simulink model "AvonGasTurbineFAult"  (R2016b)
settings: Solver=ode45  StartTime=0.0  StopTime=3000  FixedStep=1  RelTol=1e-3  EnableMultiTasking=on
InitFcn:
  | warning off
undefined symbols (not defined in the file or in its folder): flagFalut, thresholdbound, xflt
libraries: neural x74, fuzblock x6, simulink x5
(part 2 of 4)

== system AvonGasTurbineFAult/IGV/Layer 2 ==
  "a{1} " : Inport  PortDimensions=10
      mask Display: e = 0.06;c1 = [120 230 180]/255;c2 = ([120 230 180]+0)/(256+128);c3 = ([120 230 180]+128)/(256+128);patch([0 1 1 0],[0 0 1 1],c1);patch([0 1 1 1-e 1-e 0+e],[0 0 1 1-e 0+e 0+e],c2);patch([0 0 1 1-e 0+e 0+e],[0 1 1 1-e 1-e 0+e],c3);plot([0 1 1 0 0],[0 0 1 1 0]);
  Delays 1 : Subsystem
      mask Display: e = 0.06;c1 = [120 150 230]/255;c2 = ([120 150 230]+0)/383;c3 = ([120 150 230]+128)/383;patch([0 1 1 0],[0 0 1 1],c1);patch([0 1 1 1-e 1-e 0+e],[0 0 1 1-e 0+e 0+e],c2);patch([0 0 1 1-e 0+e 0+e],[0 1 1 1-e 1-e 0+e],c3);plot([0 1 1 0 0],[0 0 1 1 0]);disp('0');
  "LW{2,1}" : Subsystem
      mask Display: e = 0.06;c1 = [120 150 230]/255;c2 = ([120 150 230]+0)/383;c3 = ([120 150 230]+128)/383;patch([0 1 1 0],[0 0 1 1],c1);patch([0 1 1 1-e 1-e 0+e],[0 0 1 1-e 0+e 0+e],c2);patch([0 0 1 1-e 0+e 0+e],[0 1 1 1-e 1-e 0+e],c3);plot([0 1 1 0 0],[0 0 1 1 0]);disp('W');
  "b{2}" : Constant  Value=[-1.4853043976248173;-0.85618625825271266;-1.763034308041038;0.36633384062384799;1.9272762947772668]
      mask Display: e = 0.06;c1 = [120 150 230]/255;c2 = ([120 150 230]+0)/383;c3 = ([120 150 230]+128)/383;patch([0 1 1 0],[0 0 1 1],c1);patch([0 1 1 1-e 1-e 0+e],[0 0 1 1-e 0+e 0+e],c2);patch([0 0 1 1-e 0+e 0+e],[0 1 1 1-e 1-e 0+e],c3);plot([0 1 1 0 0],[0 0 1 1 0]);disp('b');
  netsum : Sum  Inputs=2  SaturateOnIntegerOverflow=on  InputSameDT=on  OutDataTypeStr=Inherit: Same as first input
      mask Display: e = 0.06;c1 = [120 150 230]/255;c2 = ([120 150 230]+0)/383;c3 = ([120 150 230]+128)/383;patch([0 1 1 0],[0 0 1 1],c1);patch([0 1 1 1-e 1-e 0+e],[0 0 1 1-e 0+e 0+e],c2);patch([0 0 1 1-e 0+e 0+e],[0 1 1 1-e 1-e 0+e],c3);plot([0 1 1 0 0],[0 0 1 1 0]);disp('+');
  softmax : neural/Transfer Functions/softmax
  "a{2}" : Outport  InitialOutput=[0;0;0;0;0]
      mask Display: e = 0.06;c1 = [120 230 180]/255;c2 = ([120 230 180]+0)/(256+128);c3 = ([120 230 180]+128)/(256+128);patch([0 1 1 0],[0 0 1 1],c1);patch([0 1 1 1-e 1-e 0+e],[0 0 1 1-e 0+e 0+e],c2);patch([0 0 1 1-e 0+e 0+e],[0 1 1 1-e 1-e 0+e],c3);plot([0 1 1 0 0],[0 0 1 1 0]);
  wires:
  "a{1} "/1 -> Delays 1/1("p{2}")
  Delays 1/1("pd{2,1}") -> "LW{2,1}"/1("ad{2,1}")
  "LW{2,1}"/1("lz{2,1}") -> netsum/1
  "b{2}"/1 -> netsum/2
  netsum/1 -> softmax/1
  softmax/1 -> "a{2}"/1

== system AvonGasTurbineFAult/IGV/Process Input 1 ==
  x : Inport  PortDimensions=6
      mask Display: e = 0.06;c1 = [120 230 180]/255;c2 = ([120 230 180]+0)/(256+128);c3 = ([120 230 180]+128)/(256+128);patch([0 1 1 0],[0 0 1 1],c1);patch([0 1 1 1-e 1-e 0+e],[0 0 1 1-e 0+e 0+e],c2);patch([0 0 1 1-e 0+e 0+e],[0 1 1 1-e 1-e 0+e],c3);plot([0 1 1 0 0],[0 0 1 1 0]);
  mapminmax : neural/Processing Functions/mapminmax  xmin=[-0.093008103798728925;0;-5.6896731350681762;0]  xmax=[0;20.262976664010012;-1.0691054727469123;22.645033295809071]  ymin=-1  ymax=1
  removeconstantrows : neural/Processing Functions/removeconstantrows  inputSize=6  keep=[1 3 4 5]
  p : Outport  PortDimensions=4
      mask Display: e = 0.06;c1 = [120 230 180]/255;c2 = ([120 230 180]+0)/(256+128);c3 = ([120 230 180]+128)/(256+128);patch([0 1 1 0],[0 0 1 1],c1);patch([0 1 1 1-e 1-e 0+e],[0 0 1 1-e 0+e 0+e],c2);patch([0 0 1 1-e 0+e 0+e],[0 1 1 1-e 1-e 0+e],c3);plot([0 1 1 0 0],[0 0 1 1 0]);
  wires:
  x/1 -> removeconstantrows/1
  removeconstantrows/1 -> mapminmax/1
  mapminmax/1 -> p/1

== system AvonGasTurbineFAult/IGV/Process Output 1 ==
  a : Inport  PortDimensions=5
      mask Display: e = 0.06;c1 = [120 230 180]/255;c2 = ([120 230 180]+0)/(256+128);c3 = ([120 230 180]+128)/(256+128);patch([0 1 1 0],[0 0 1 1],c1);patch([0 1 1 1-e 1-e 0+e],[0 0 1 1-e 0+e 0+e],c2);patch([0 0 1 1-e 0+e 0+e],[0 1 1 1-e 1-e 0+e],c3);plot([0 1 1 0 0],[0 0 1 1 0]);
  y : Outport  PortDimensions=5
      mask Display: e = 0.06;c1 = [120 230 180]/255;c2 = ([120 230 180]+0)/(256+128);c3 = ([120 230 180]+128)/(256+128);patch([0 1 1 0],[0 0 1 1],c1);patch([0 1 1 1-e 1-e 0+e],[0 0 1 1-e 0+e 0+e],c2);patch([0 0 1 1-e 0+e 0+e],[0 1 1 1-e 1-e 0+e],c3);plot([0 1 1 0 0],[0 0 1 1 0]);
  wires:
  a/1 -> y/1

== system AvonGasTurbineFAult/Subsystem/Combustor ==
  FG temp : Inport
  FG flow : Inport  Port=2
  FG press : Inport  Port=3
  air_flow : Inport  Port=4
  air temp : Inport  Port=5
  air_press : Inport  Port=6
  Scope1 : Scope
  Scope2 : Scope
  Scope3 : Scope
  combustion chamber 1 : Subsystem
  cooling_air_temp : Outport
  flow_chamber : Outport  Port=2
  temp_chamber : Outport  Port=3
  press_hot_gas : Outport  Port=4
  wires:
  FG flow/1 -> combustion chamber 1/1(Fg flow)
  FG press/1 -> combustion chamber 1/2(FG press)
  FG temp/1 -> combustion chamber 1/3(FG temp)
  combustion chamber 1/1(temp chamber 1) -> Scope1/1, temp_chamber/1
  air_press/1 -> combustion chamber 1/6(air_press)
  air temp/1 -> Scope2/1, cooling_air_temp/1, combustion chamber 1/5(air_temp)
  combustion chamber 1/2(flow) -> Scope3/1, flow_chamber/1
  air_flow/1 -> combustion chamber 1/4(air flow)
  combustion chamber 1/3(Gas_press) -> press_hot_gas/1

== system AvonGasTurbineFAult/Subsystem/FG MCV model ==
  FG CV pos (%) chmb1 : Inport
  main FG line prss : Inport  Port=2
  FG temp. : Inport  Port=3
  " Memory " : Memory  X0=1.9
  CV model chamber 2 : Subsystem
  Subsystem1 : Subsystem
  FG Temp (oC) : Outport
  FG Flow @bur (kg/s) : Outport  Port=2
  FG pr @bur (kPa) : Outport  Port=3
  FG skid inlet prss (kPa) : Outport  Port=4
  tag scope: FG_flow=global
  wires:
  Subsystem1/2(skid temp) -> CV model chamber 2/3(FG temp.)
  " Memory "/1 -> Subsystem1/3(FG flow)
  main FG line prss/1 -> Subsystem1/1(gas prss)
  Subsystem1/1(" FG skid inlet prss") -> CV model chamber 2/2(Skid inlet prss), FG skid inlet prss (kPa)/1
  FG temp./1 -> Subsystem1/2(FG temp.), FG Temp (oC)/1
  CV model chamber 2/1(FG pr @bur) -> FG pr @bur (kPa)/1
  FG CV pos (%) chmb1/1 -> CV model chamber 2/1(FG valve pos.)
  CV model chamber 2/2(FG flow) -> FG Flow @bur (kg/s)/1, [FG_flow], " Memory "/1

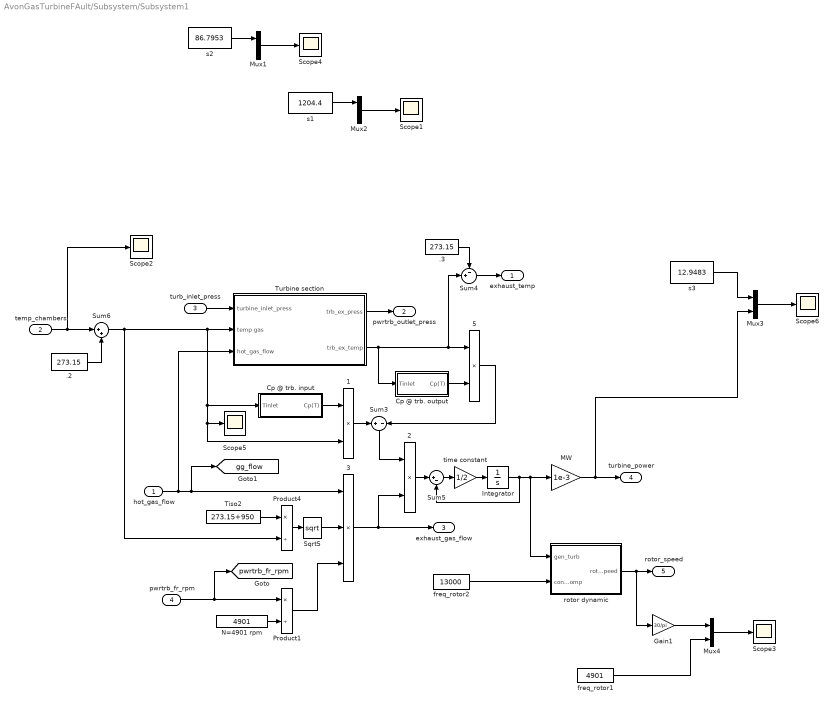
== system AvonGasTurbineFAult/Subsystem/Subsystem1 ==
  hot_gas_flow : Inport
  temp_chambers : Inport  Port=2
  turb_inlet_press : Inport  Port=3
  pwrtrb_fr_rpm : Inport  Port=4
  "    .2" : Constant  Value=273.15
  "    .3" : Constant  Value=273.15
  " 1" : Product  RndMeth=Zero
  " 2" : Product  RndMeth=Zero
  " 3" : Product  Inputs=3  RndMeth=Zero
  " 5" : Product  RndMeth=Zero
  Cp @ trb. input : Subsystem
  Cp @ trb. output : Subsystem
  Gain1 : Gain  Gain=30/pi
  Integrator : Integrator  InitialCondition=13000  LimitOutput=on  UpperSaturationLimit=20000  LowerSaturationLimit=1
  MW : Gain  Gain=1e-3
  Mux1 : Mux  Inputs=2
  Mux2 : Mux  Inputs=3
  Mux3 : Mux  Inputs=2
  Mux4 : Mux  Inputs=2
  N=4901 rpm : Constant  Value=4901
  Product1 : Product  Inputs=*/  RndMeth=Zero
  Product4 : Product  Inputs=*/  RndMeth=Zero
  Scope{1..6} (6 alike) : Scope
  Sqrt5 : Sqrt  SaturateOnIntegerOverflow=on
  Sum3 : Sum  Inputs=+-
  Sum4 : Sum  Inputs=-+|
  Sum5 : Sum  Inputs=|+-
  Sum6 : Sum  Inputs=|++
  Tiso2 : Constant  Value=273.15+950
  Turbine section : Subsystem
  freq_rotor1 : Constant  Value=4901
  freq_rotor2 : Constant  Value=13000
  rotor dynamic : Subsystem
  s1 : Constant  Value=1204.4
  s2 : Constant  Value=86.7953
  s3 : Constant  Value=12.9483
  time constant : Gain  Gain=1/2
  exhaust_temp : Outport
  pwrtrb_outlet_press : Outport  Port=2
  exhaust_gas_flow : Outport  Port=3
  turbine_power : Outport  Port=4
  rotor_speed : Outport  Port=5
  tag scope: gg_flow=global, pwrtrb_fr_rpm=global
  wires:
  Turbine section/2(trb_ex_temp) -> " 5"/1, Sum4/2, Cp @ trb. output/1(Tinlet)
  s3/1 -> Mux3/1
  Mux3/1 -> Scope6/1
  turb_inlet_press/1 -> Turbine section/1(turbine_inlet_press)
  "    .3"/1 -> Sum4/1
  Sum4/1 -> exhaust_temp/1
  temp_chambers/1 -> Scope2/1, Sum6/1
  "    .2"/1 -> Sum6/2
  s1/1 -> Mux2/1
  Mux2/1 -> Scope1/1
  s2/1 -> Mux1/1
  Mux1/1 -> Scope4/1
  " 2"/1 -> Sum5/1
  " 5"/1 -> Sum3/2
  Cp @ trb. output/1(Cp(T)) -> " 5"/2
  Cp @ trb. input/1(Cp(T)) -> " 1"/1
  time constant/1 -> Integrator/1
  Sum5/1 -> time constant/1
  " 1"/1 -> Sum3/1
  Sum3/1 -> " 2"/1
  Tiso2/1 -> Product4/1
  Sum6/1 -> Product4/2, Cp @ trb. input/1(Tinlet), " 1"/2, Scope5/1, Turbine section/2(temp gas)
  Product4/1 -> Sqrt5/1
  N=4901 rpm/1 -> Product1/2
  pwrtrb_fr_rpm/1 -> [pwrtrb_fr_rpm], Product1/1
  Product1/1 -> " 3"/3
  Sqrt5/1 -> " 3"/2
  hot_gas_flow/1 -> Turbine section/3(hot_gas_flow), [gg_flow], " 3"/1
  " 3"/1 -> exhaust_gas_flow/1, " 2"/2
  Turbine section/1(trb_ex_press) -> pwrtrb_outlet_press/1
  rotor dynamic/1(rotor_speed) -> Gain1/1, rotor_speed/1
  Integrator/1 -> Sum5/2, MW/1, rotor dynamic/1(gen_turb)
  MW/1 -> turbine_power/1, Mux3/2
  Mux4/1 -> Scope3/1
  freq_rotor1/1 -> Mux4/2
  Gain1/1 -> Mux4/1
  freq_rotor2/1 -> rotor dynamic/2(consm_comp)

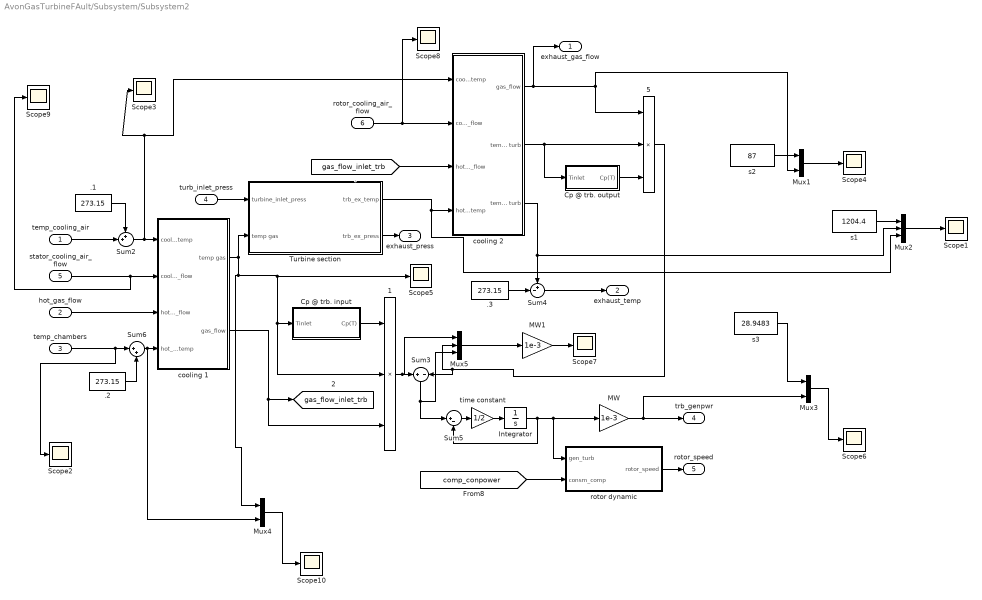
== system AvonGasTurbineFAult/Subsystem/Subsystem2 ==
  temp_cooling_air : Inport
  hot_gas_flow : Inport  Port=2
  temp_chambers : Inport  Port=3
  turb_inlet_press : Inport  Port=4
  stator_cooling_air_flow : Inport  Port=5
  rotor_cooling_air_flow : Inport  Port=6
  "    .1" : Constant  Value=273.15
  "    .2" : Constant  Value=273.15
  "    .3" : Constant  Value=273.15
  " 1" : Product  Inputs=3  RndMeth=Zero
  " 5" : Product  Inputs=3  RndMeth=Zero
  Cp @ trb. input : Subsystem
  Cp @ trb. output : Subsystem
  Integrator : Integrator  InitialCondition=13500  LimitOutput=on  UpperSaturationLimit=34000  LowerSaturationLimit=10
  MW : Gain  Gain=1e-3
  MW1 : Gain  Gain=1e-3
  Mux1 : Mux  Inputs=2
  Mux2 : Mux  Inputs=3
  Mux3 : Mux  Inputs=2
  Mux4 : Mux  Inputs=2
  Mux5 : Mux  Inputs=3
  Scope{1..10} (10 alike) : Scope
  Sum2 : Sum  Inputs=++|
  Sum3 : Sum  Inputs=+-
  Sum4 : Sum  Inputs=+-|
  Sum5 : Sum  Inputs=|+-
  Sum6 : Sum  Inputs=|++
  Turbine section : Subsystem
  cooling 1 : Subsystem
  cooling 2 : Subsystem
  "rotor dynamic " : Subsystem
  s1 : Constant  Value=1204.4
  s2 : Constant  Value=87
  s3 : Constant  Value=28.9483
  time constant : Gain  Gain=1/2
  exhaust_gas_flow : Outport
  exhaust_temp : Outport  Port=2
  exhaust_press : Outport  Port=3
  trb_genpwr : Outport  Port=4
  rotor_speed : Outport  Port=5
  tag scope: gas_flow_inlet_trb=global
  wires:
  Sum2/1 -> cooling 1/1(cooling_air_temp), cooling 2/1(cooling_air_temp), Scope3/1
  hot_gas_flow/1 -> cooling 1/3(hot_gas_flow)
  " 1"/1 -> Mux5/1, Sum3/1
  rotor_cooling_air_flow/1 -> Scope8/1, cooling 2/2(cooling_air_flow)
  Sum5/1 -> time constant/1
  time constant/1 -> Integrator/1
  [gas_flow_inlet_trb] -> cooling 2/3(hot_gas_flow)
  Cp @ trb. input/1(Cp(T)) -> " 1"/1
  Turbine section/1(trb_ex_temp) -> Mux2/3, cooling 2/4(hot_gas_temp)
  cooling 2/3(temp exh turb) -> Mux2/2, Sum4/1
  Cp @ trb. output/1(Cp(T)) -> " 5"/3
  " 5"/1 -> Sum3/2, Mux5/2
  cooling 1/2(gas_flow) -> " 1"/3, [gas_flow_inlet_trb]
  Sum3/1 -> Mux5/3, Sum5/1
  Mux1/1 -> Scope4/1
  s2/1 -> Mux1/1
  cooling 2/1(gas_flow) -> " 5"/1, Mux1/2, exhaust_gas_flow/1
  Mux2/1 -> Scope1/1
  s1/1 -> Mux2/1
  "    .1"/1 -> Sum2/1
  temp_cooling_air/1 -> Sum2/2
  "    .2"/1 -> Sum6/2
  temp_chambers/1 -> Scope2/1, Sum6/1
  Sum4/1 -> exhaust_temp/1
  "    .3"/1 -> Sum4/2
  turb_inlet_press/1 -> Turbine section/1(turbine_inlet_press)
  Mux3/1 -> Scope6/1
  s3/1 -> Mux3/1
  Integrator/1 -> "rotor dynamic "/1(gen_turb), MW/1, Sum5/2
  cooling 2/2(temp turb) -> Cp @ trb. output/1(Tinlet), " 5"/2
  Turbine section/2(trb_ex_press) -> exhaust_press/1
  MW/1 -> Mux3/2, trb_genpwr/1
  [comp_conpower] -> "rotor dynamic "/2(consm_comp)
  "rotor dynamic "/1(rotor_speed) -> rotor_speed/1
  stator_cooling_air_flow/1 -> cooling 1/2(cooling_air_flow), Scope9/1
  Mux4/1 -> Scope10/1
  cooling 1/1(temp gas) -> Turbine section/2(temp gas), Cp @ trb. input/1(Tinlet), " 1"/2, Scope5/1, Mux4/1
  Sum6/1 -> Mux4/2, cooling 1/4(hot_gas_temp)
  Mux5/1 -> MW1/1
  MW1/1 -> Scope7/1

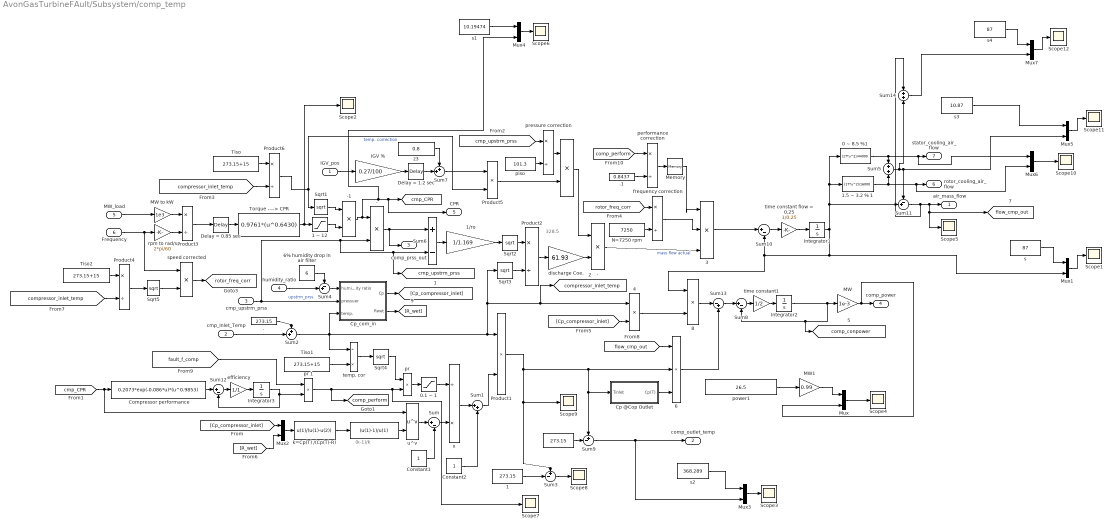
== system AvonGasTurbineFAult/Subsystem/comp_temp ==
  note: (k-1)/k
  note: 328.5
  IGV_pos : Inport
  cmp_Inlet_Temp : Inport  Port=2
  cmp_upstrm_prss : Inport  Port=3
  humidity_ratio : Inport  Port=4
  MW_load : Inport  Port=5
  Frequency : Inport  Port=6
  " " : Fcn  Expr=(u(1)-1)/u(1)
  "    " : Constant  Value=273.15
  "     " : Product  RndMeth=Zero
  "    1" : Constant  Value=273.15
  " 1.5 ~ 3.2 % 1" : Fcn  Expr=(17*u^2)/16000  SampleTime=1
  " 3" : Product  Inputs=3  RndMeth=Zero
  " 4" : Product  RndMeth=Zero
  " 6" : Product  Inputs=3  RndMeth=Zero
  " 8" : Product  RndMeth=Zero
  - : Product  RndMeth=Zero
  -1 : Product  RndMeth=Zero
  . : Constant  Value=273.15
  ". " : Product  RndMeth=Zero
  .1 : Constant  Value=0.8437
  0 ~ 8.5 %1 : Fcn  Expr=(17*u^2)/44000  SampleTime=1
  0.1 ~ 1 : Saturate  UpperLimit=1  LowerLimit=0.1
  1 ~ 12 : Saturate  UpperLimit=20  LowerLimit=1
  1/ro : Gain  Gain=1/1.169
  6% humidity drop in air filter : Constant  Value=6
  "Compressor performance " : Fcn  Expr=0.2073*exp(-0.086*u)*(u^0.9853)
  Constant1 : Constant
  Constant2 : Constant
  Cp @Cop Outlet : Subsystem
  Cp_com_in : Subsystem
  Delay = 0.85 sec : TransportDelay  DelayTime=0.85  InitialOutput=10.706
  Delay = 1.2 sec : TransportDelay  DelayTime=1.2  InitialOutput=0.27
  IGV % : Gain  Gain=0.27/100
  Integrator1 : Integrator  InitialCondition=87  LimitOutput=on  UpperSaturationLimit=140  LowerSaturationLimit=1
  Integrator2 : Integrator  InitialCondition=28000  LimitOutput=on  UpperSaturationLimit=32000  LowerSaturationLimit=10
  Integrator3 : Integrator  InitialCondition=0.6  LimitOutput=on  UpperSaturationLimit=1  LowerSaturationLimit=0
  MW : Gain  Gain=1e-3
  MW to kW : Gain  Gain=1e3
  MW1 : Gain  Gain=0.99
  Memory : Memory  X0=1.5
  Mux{,1..7} (8 alike) : Mux  Inputs=2
  N=7250 rpm : Constant  Value=7250
  Product1 : Product  RndMeth=Zero
  Product{2..4,6} (4 alike) : Product  Inputs=*/  RndMeth=Zero
  Product5 : Product  RndMeth=Zero
  Scope{1..12} (12 alike) : Scope
  Sqrt{1..5} (5 alike) : Sqrt  SaturateOnIntegerOverflow=on
  Sum{,8,10,12} (4 alike) : Sum  Inputs=|+-
  Sum1 : Sum  Inputs=|++
  Sum11 : Sum  Inputs=-+|
  Sum13 : Sum  Inputs=|-+
  Sum14 : Sum
  Sum2 : Sum  Inputs=++|
  Sum3 : Sum  Inputs=+-|
  Sum4 : Sum  Inputs=-+|
  Sum5 : Sum
  Sum6 : Sum  Inputs=+-
  Sum7 : Sum  Inputs=++|
  Sum9 : Sum  Inputs=+-|
  Tiso : Constant  Value=273.15+15
  Tiso1 : Constant  Value=273.15+15
  Tiso2 : Constant  Value=273.15+15
  Torque ----> CPR : Fcn  Expr=0.9761*(u^0.6430)
  "discharge Coe. " : Gain  Gain=61.93
  efficiency : Gain  Gain=1/1
  frequency correction : Product  Inputs=*/  RndMeth=Zero
  k=Cp(T) /(Cp(T)-R) : Fcn  Expr=u(1)/(u(1)-u(2))
  performance correction : Product  Inputs=*/  RndMeth=Zero
  piso : Constant  Value=101.3
  power1 : Constant  Value=26.5
  "pr " : Product  RndMeth=Zero
  pr 1 : Product  RndMeth=Zero
  pressure correction : Product  Inputs=*/  RndMeth=Zero
  rpm to rad/s : Gain  Gain=2*pi/60
  s : Constant  Value=87
  s1 : Constant  Value=10.19474
  s2 : Constant  Value=368.289
  s3 : Constant  Value=10.87
  s4 : Constant  Value=87
  speed corrected : Product  RndMeth=Zero
  temp. cor : Product  Inputs=/*  RndMeth=Zero
  time constant flow = 0.25 : Gain  Gain=1/0.25
  time constant1 : Gain  Gain=1/2
  u^v : Math  Operator=pow  SaturateOnIntegerOverflow=on
  x : Product  Inputs=/*  RndMeth=Zero
  z3 : Constant  Value=0.8
  air_mass_flow : Outport
  comp_outlet_temp : Outport  Port=2
  comp_prss_out : Outport  Port=3
  comp_power : Outport  Port=4
  CPR : Outport  Port=5
  rotor_cooling_air_flow : Outport  Port=6
  stator_cooling_air_flow : Outport  Port=7
  tag scope: cmp_CPR=global, cmp_upstrm_prss=global, comp_conpower=global, comp_perform=global, compressor_inlet_temp=global, flow_cmp_out=global, rotor_freq_corr=global
  wires:
  [cmp_CPR] -> "Compressor performance "/1, u^v/1
  " "/1 -> u^v/2
  u^v/1 -> Sum/1
  Sum/1 -> x/2
  Constant2/1 -> Sum1/2
  Sum1/1 -> Product1/2
  Sum2/1 -> Cp_com_in/3(temp.), Product1/1, Sqrt3/1, [compressor_inlet_temp], " 4"/1, temp. cor/1
  x/1 -> Sum1/1
  Constant1/1 -> Sum/2
  cmp_upstrm_prss/1 -> Cp_com_in/2(pressuer), -/2, Sum6/2, [cmp_upstrm_prss]  "upstrm_prss"
  cmp_Inlet_Temp/1 -> Sum2/2
  "Compressor performance "/1 -> Sum12/1
  0.1 ~ 1/1 -> x/1
  k=Cp(T) /(Cp(T)-R)/1 -> " "/1
  Cp_com_in/1(Cp) -> [Cp_compressor_inlet]
  Sum4/1 -> Cp_com_in/1(humidity ratio)
  humidity_ratio/1 -> Sum4/2
  6% humidity drop in air filter/1 -> Sum4/1
  -/1 -> comp_prss_out/1, Sum6/1
  Frequency/1 -> speed corrected/1, rpm to rad/s/1
  Sum6/1 -> 1/ro/1
  1/ro/1 -> Sqrt2/1
  Sqrt3/1 -> Product2/2
  Product2/1 -> "discharge Coe. "/1
  Sqrt2/1 -> Product2/1
  IGV_pos/1 -> IGV %/1
  piso/1 -> pressure correction/2
  [cmp_upstrm_prss] -> pressure correction/1
  Product5/1 -> "     "/2
  "discharge Coe. "/1 -> ". "/2
  "     "/1 -> ". "/1
  ". "/1 -> " 3"/3  "mass flow actual"
  Product6/1 -> Product5/2, Sqrt1/1  "temp. correction"
  Tiso/1 -> Product6/1
  [compressor_inlet_temp] -> Product6/2
  pressure correction/1 -> "     "/1
  1 ~ 12/1 -> -1/2
  N=7250 rpm/1 -> frequency correction/2
  [rotor_freq_corr] -> frequency correction/1
  frequency correction/1 -> " 3"/2
  " 3"/1 -> Sum10/1
  [Cp_compressor_inlet] -> " 4"/2
  Sum10/1 -> time constant flow = 0.25/1
  time constant flow = 0.25/1 -> Integrator1/1
  " 4"/1 -> " 8"/2
  " 8"/1 -> Sum13/1
  Sqrt1/1 -> -1/1
  Sum7/1 -> Product5/1
  z3/1 -> Sum7/1
  IGV %/1 -> Delay = 1.2 sec/1
  Delay = 1.2 sec/1 -> Sum7/2
  MW_load/1 -> MW to kW/1
  Cp_com_in/2(Rwet) -> [R_wet]
  Mux2/1 -> k=Cp(T) /(Cp(T)-R)/1
  [Cp_compressor_inlet] -> Mux2/1
  [R_wet] -> Mux2/2
  Sum8/1 -> time constant1/1
  time constant1/1 -> Integrator2/1
  Sum13/1 -> Sum8/1
  ./1 -> Sum2/1
  Tiso1/1 -> temp. cor/2
  temp. cor/1 -> Sqrt4/1
  "pr "/1 -> 0.1 ~ 1/1
  Sum12/1 -> efficiency/1
  efficiency/1 -> Integrator3/1
  Sqrt4/1 -> "pr "/1
  Torque ----> CPR/1 -> 1 ~ 12/1, Scope2/1
  MW to kW/1 -> Product3/1
  rpm to rad/s/1 -> Product3/2
  Integrator3/1 -> pr 1/2, Sum12/2
  Integrator2/1 -> MW/1, [comp_conpower], Sum8/2
  Product1/1 -> " 6"/2, Cp @Cop Outlet/1(Tinlet), Sum9/1, Scope9/1, Sum3/1
  Cp @Cop Outlet/1(Cp(T)) -> " 6"/3
  " 6"/1 -> Sum13/2
  "    "/1 -> Sum9/2
  Tiso2/1 -> Product4/1
  [compressor_inlet_temp] -> Product4/2
  speed corrected/1 -> [rotor_freq_corr]
  Product4/1 -> Sqrt5/1
  Sqrt5/1 -> speed corrected/2
  [flow_cmp_out] -> " 6"/1
  Mux/1 -> Scope4/1
  Sum11/1 -> Sum14/1, Scope5/1, [flow_cmp_out], air_mass_flow/1
  0 ~ 8.5 %1/1 -> Sum5/1, Mux6/1, stator_cooling_air_flow/1
  Integrator1/1 -> Mux1/2, " 8"/1, Sum10/2, Sum11/2, " 1.5 ~ 3.2 % 1"/1, 0 ~ 8.5 %1/1
  Mux1/1 -> Scope1/1
  s/1 -> Mux1/1
  Product3/1 -> Delay = 0.85 sec/1
  Delay = 0.85 sec/1 -> Torque ----> CPR/1
  power1/1 -> MW1/1
  Mux3/1 -> Scope3/1
  s2/1 -> Mux3/1
  MW/1 -> Mux/2, comp_power/1
  Mux4/1 -> Scope6/1
  s1/1 -> Mux4/1
  -1/1 -> -/1, Mux4/2, [cmp_CPR], CPR/1
  Sum9/1 -> Mux3/2, comp_outlet_temp/1
  "    1"/1 -> Sum3/2
  Sum3/1 -> Scope8/1
  MW1/1 -> Mux/1
  Sum5/1 -> Sum14/2, Sum11/1, Mux5/2
  Mux5/1 -> Scope11/1
  s3/1 -> Mux5/1
  Mux6/1 -> Scope10/1
  " 1.5 ~ 3.2 % 1"/1 -> Sum5/2, Mux6/2, rotor_cooling_air_flow/1
  Sum14/1 -> Mux7/2
  Mux7/1 -> Scope12/1
  s4/1 -> Mux7/1
  pr 1/1 -> [comp_perform], "pr "/2, Scope7/1
  [fault_f_comp] -> pr 1/1
  performance correction/1 -> Memory/1
  .1/1 -> performance correction/2
  [comp_perform] -> performance correction/1
  Memory/1 -> " 3"/1

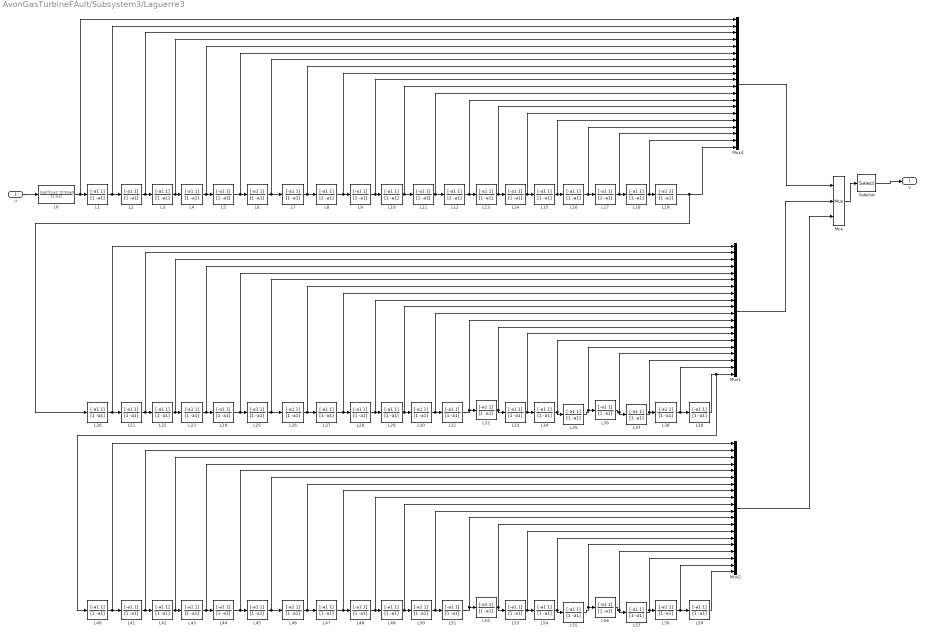
== system AvonGasTurbineFAult/Subsystem3/Laguerre3 ==
  u : Inport
  L0 : DiscreteTransferFcn  Numerator=[sqrt((1-a1^2)*smp)]  Denominator=[1 -a1]  SampleTime=smp  StateIdentifier=L0
  L{1..59} (59 alike) : DiscreteTransferFcn  Numerator=[-a1 1]  Denominator=[1 -a1]  SampleTime=smp  StateIdentifier=L1
  Mux : Mux  Inputs=3
  Mux1 : Mux  Inputs=20
  Mux2 : Mux  Inputs=20
  Mux4 : Mux  Inputs=20
  Selector : Selector  InputPortWidth=60  IndexOptions=Index vector (dialog)  Indices=1:fltrordr  OutputSizes=1
  v : Outport
  wires:
  Mux2/1 -> Mux/3
  L59/1 -> Mux2/20
  L58/1 -> L59/1, Mux2/19
  L57/1 -> L58/1, Mux2/18
  L56/1 -> L57/1, Mux2/17
  L55/1 -> L56/1, Mux2/16
  L54/1 -> L55/1, Mux2/15
  L53/1 -> L54/1, Mux2/14
  L52/1 -> L53/1, Mux2/13
  L51/1 -> L52/1, Mux2/12
  L50/1 -> L51/1, Mux2/11
  L49/1 -> L50/1, Mux2/10
  L48/1 -> L49/1, Mux2/9
  L47/1 -> L48/1, Mux2/8
  L46/1 -> L47/1, Mux2/7
  L45/1 -> L46/1, Mux2/6
  L44/1 -> L45/1, Mux2/5
  L43/1 -> L44/1, Mux2/4
  L42/1 -> L43/1, Mux2/3
  L41/1 -> L42/1, Mux2/2
  L40/1 -> L41/1, Mux2/1
  Selector/1 -> v/1
  Mux4/1 -> Mux/1
  Mux/1 -> Selector/1
  Mux1/1 -> Mux/2
  L39/1 -> Mux1/20, L40/1
  L38/1 -> Mux1/19, L39/1
  L37/1 -> Mux1/18, L38/1
  L36/1 -> Mux1/17, L37/1
  L35/1 -> Mux1/16, L36/1
  L34/1 -> Mux1/15, L35/1
  L33/1 -> Mux1/14, L34/1
  L32/1 -> Mux1/13, L33/1
  L31/1 -> Mux1/12, L32/1
  L30/1 -> Mux1/11, L31/1
  L29/1 -> Mux1/10, L30/1
  L28/1 -> Mux1/9, L29/1
  L27/1 -> Mux1/8, L28/1
  L26/1 -> Mux1/7, L27/1
  L25/1 -> Mux1/6, L26/1
  L24/1 -> Mux1/5, L25/1
  L23/1 -> Mux1/4, L24/1
  L22/1 -> Mux1/3, L23/1
  L21/1 -> Mux1/2, L22/1
  L20/1 -> Mux1/1, L21/1
  L19/1 -> L20/1, Mux4/20
  L18/1 -> Mux4/19, L19/1
  L17/1 -> Mux4/18, L18/1
  L16/1 -> Mux4/17, L17/1
  L15/1 -> Mux4/16, L16/1
  L14/1 -> Mux4/15, L15/1
  L13/1 -> Mux4/14, L14/1
  L12/1 -> Mux4/13, L13/1
  L11/1 -> Mux4/12, L12/1
  L10/1 -> Mux4/11, L11/1
  L9/1 -> Mux4/10, L10/1
  L8/1 -> Mux4/9, L9/1
  u/1 -> L0/1
  L7/1 -> Mux4/8, L8/1
  L6/1 -> L7/1, Mux4/7
  L5/1 -> L6/1, Mux4/6
  L0/1 -> Mux4/1, L1/1
  L4/1 -> L5/1, Mux4/5
  L3/1 -> L4/1, Mux4/4
  L2/1 -> L3/1, Mux4/3
  L1/1 -> L2/1, Mux4/2

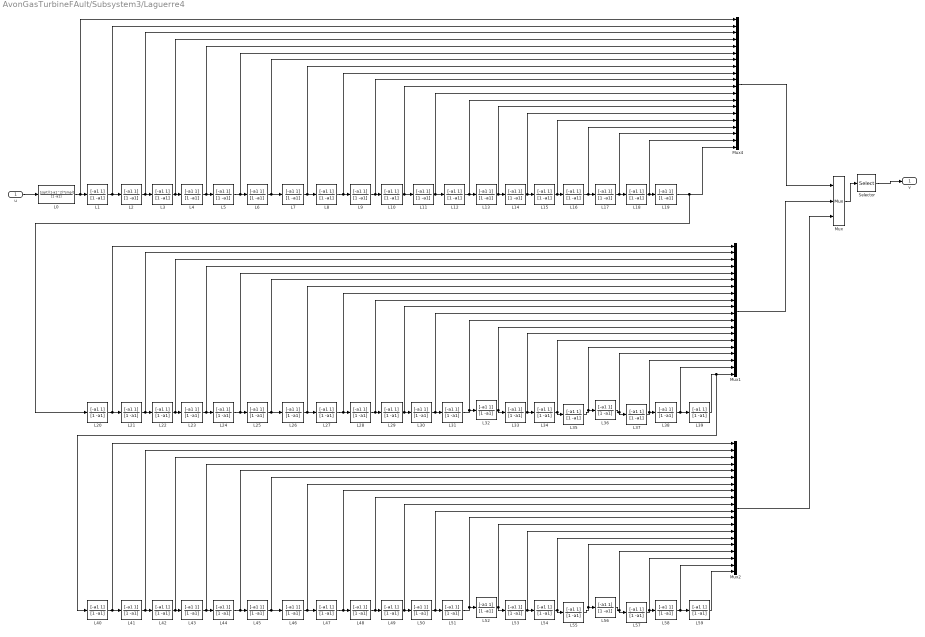
== system AvonGasTurbineFAult/Subsystem3/Laguerre4 ==
  u : Inport
  L0 : DiscreteTransferFcn  Numerator=[sqrt((1-a1^2)*smp)]  Denominator=[1 -a1]  SampleTime=smp  StateIdentifier=L0
  L{1..59} (59 alike) : DiscreteTransferFcn  Numerator=[-a1 1]  Denominator=[1 -a1]  SampleTime=smp  StateIdentifier=L1
  Mux : Mux  Inputs=3
  Mux1 : Mux  Inputs=20
  Mux2 : Mux  Inputs=20
  Mux4 : Mux  Inputs=20
  Selector : Selector  InputPortWidth=60  IndexOptions=Index vector (dialog)  Indices=1:fltrordr  OutputSizes=1
  v : Outport
  wires:
  L1/1 -> Mux4/2, L2/1
  L2/1 -> Mux4/3, L3/1
  L3/1 -> Mux4/4, L4/1
  L4/1 -> Mux4/5, L5/1
  L0/1 -> L1/1, Mux4/1
  L5/1 -> Mux4/6, L6/1
  L6/1 -> Mux4/7, L7/1
  L7/1 -> L8/1, Mux4/8
  u/1 -> L0/1
  L8/1 -> L9/1, Mux4/9
  L9/1 -> L10/1, Mux4/10
  L10/1 -> L11/1, Mux4/11
  L11/1 -> L12/1, Mux4/12
  L12/1 -> L13/1, Mux4/13
  L13/1 -> L14/1, Mux4/14
  L14/1 -> L15/1, Mux4/15
  L15/1 -> L16/1, Mux4/16
  L16/1 -> L17/1, Mux4/17
  L17/1 -> L18/1, Mux4/18
  L18/1 -> L19/1, Mux4/19
  L19/1 -> Mux4/20, L20/1
  L20/1 -> L21/1, Mux1/1
  L21/1 -> L22/1, Mux1/2
  L22/1 -> L23/1, Mux1/3
  L23/1 -> L24/1, Mux1/4
  L24/1 -> L25/1, Mux1/5
  L25/1 -> L26/1, Mux1/6
  L26/1 -> L27/1, Mux1/7
  L27/1 -> L28/1, Mux1/8
  L28/1 -> L29/1, Mux1/9
  L29/1 -> L30/1, Mux1/10
  L30/1 -> L31/1, Mux1/11
  L31/1 -> L32/1, Mux1/12
  L32/1 -> L33/1, Mux1/13
  L33/1 -> L34/1, Mux1/14
  L34/1 -> L35/1, Mux1/15
  L35/1 -> L36/1, Mux1/16
  L36/1 -> L37/1, Mux1/17
  L37/1 -> L38/1, Mux1/18
  L38/1 -> L39/1, Mux1/19
  L39/1 -> L40/1, Mux1/20
  Mux1/1 -> Mux/2
  Mux/1 -> Selector/1
  Mux4/1 -> Mux/1
  Selector/1 -> v/1
  L40/1 -> Mux2/1, L41/1
  L41/1 -> Mux2/2, L42/1
  L42/1 -> Mux2/3, L43/1
  L43/1 -> Mux2/4, L44/1
  L44/1 -> Mux2/5, L45/1
  L45/1 -> Mux2/6, L46/1
  L46/1 -> Mux2/7, L47/1
  L47/1 -> Mux2/8, L48/1
  L48/1 -> Mux2/9, L49/1
  L49/1 -> Mux2/10, L50/1
  L50/1 -> Mux2/11, L51/1
  L51/1 -> Mux2/12, L52/1
  L52/1 -> Mux2/13, L53/1
  L53/1 -> Mux2/14, L54/1
  L54/1 -> Mux2/15, L55/1
  L55/1 -> Mux2/16, L56/1
  L56/1 -> Mux2/17, L57/1
  L57/1 -> Mux2/18, L58/1
  L58/1 -> Mux2/19, L59/1
  L59/1 -> Mux2/20
  Mux2/1 -> Mux/3

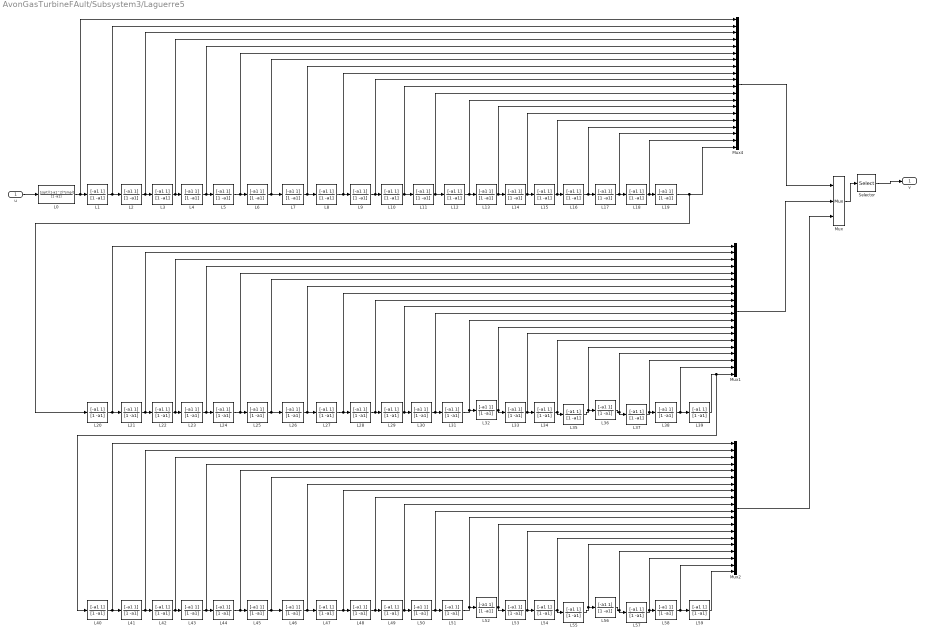
== system AvonGasTurbineFAult/Subsystem3/Laguerre5 ==
  u : Inport
  L0 : DiscreteTransferFcn  Numerator=[sqrt((1-a1^2)*smp)]  Denominator=[1 -a1]  SampleTime=smp  StateIdentifier=L0
  L{1..59} (59 alike) : DiscreteTransferFcn  Numerator=[-a1 1]  Denominator=[1 -a1]  SampleTime=smp  StateIdentifier=L1
  Mux : Mux  Inputs=3
  Mux1 : Mux  Inputs=20
  Mux2 : Mux  Inputs=20
  Mux4 : Mux  Inputs=20
  Selector : Selector  InputPortWidth=60  IndexOptions=Index vector (dialog)  Indices=1:fltrordr  OutputSizes=1
  v : Outport
  wires:
  Mux2/1 -> Mux/3
  L59/1 -> Mux2/20
  L58/1 -> L59/1, Mux2/19
  L57/1 -> L58/1, Mux2/18
  L56/1 -> L57/1, Mux2/17
  L55/1 -> L56/1, Mux2/16
  L54/1 -> L55/1, Mux2/15
  L53/1 -> L54/1, Mux2/14
  L52/1 -> L53/1, Mux2/13
  L51/1 -> L52/1, Mux2/12
  L50/1 -> L51/1, Mux2/11
  L49/1 -> L50/1, Mux2/10
  L48/1 -> L49/1, Mux2/9
  L47/1 -> L48/1, Mux2/8
  L46/1 -> L47/1, Mux2/7
  L45/1 -> L46/1, Mux2/6
  L44/1 -> L45/1, Mux2/5
  L43/1 -> L44/1, Mux2/4
  L42/1 -> L43/1, Mux2/3
  L41/1 -> L42/1, Mux2/2
  L40/1 -> L41/1, Mux2/1
  Selector/1 -> v/1
  Mux4/1 -> Mux/1
  Mux/1 -> Selector/1
  Mux1/1 -> Mux/2
  L39/1 -> Mux1/20, L40/1
  L38/1 -> Mux1/19, L39/1
  L37/1 -> Mux1/18, L38/1
  L36/1 -> Mux1/17, L37/1
  L35/1 -> Mux1/16, L36/1
  L34/1 -> Mux1/15, L35/1
  L33/1 -> Mux1/14, L34/1
  L32/1 -> Mux1/13, L33/1
  L31/1 -> Mux1/12, L32/1
  L30/1 -> Mux1/11, L31/1
  L29/1 -> Mux1/10, L30/1
  L28/1 -> Mux1/9, L29/1
  L27/1 -> Mux1/8, L28/1
  L26/1 -> Mux1/7, L27/1
  L25/1 -> Mux1/6, L26/1
  L24/1 -> Mux1/5, L25/1
  L23/1 -> Mux1/4, L24/1
  L22/1 -> Mux1/3, L23/1
  L21/1 -> Mux1/2, L22/1
  L20/1 -> Mux1/1, L21/1
  L19/1 -> L20/1, Mux4/20
  L18/1 -> Mux4/19, L19/1
  L17/1 -> Mux4/18, L18/1
  L16/1 -> Mux4/17, L17/1
  L15/1 -> Mux4/16, L16/1
  L14/1 -> Mux4/15, L15/1
  L13/1 -> Mux4/14, L14/1
  L12/1 -> Mux4/13, L13/1
  L11/1 -> Mux4/12, L12/1
  L10/1 -> Mux4/11, L11/1
  L9/1 -> Mux4/10, L10/1
  L8/1 -> Mux4/9, L9/1
  u/1 -> L0/1
  L7/1 -> Mux4/8, L8/1
  L6/1 -> L7/1, Mux4/7
  L5/1 -> L6/1, Mux4/6
  L0/1 -> Mux4/1, L1/1
  L4/1 -> L5/1, Mux4/5
  L3/1 -> L4/1, Mux4/4
  L2/1 -> L3/1, Mux4/3
  L1/1 -> L2/1, Mux4/2

== system AvonGasTurbineFAult/comp performance/Layer 1 ==
  "p{1}" : Inport  PortDimensions=6
      mask Display: e = 0.06;c1 = [120 230 180]/255;c2 = ([120 230 180]+0)/(256+128);c3 = ([120 230 180]+128)/(256+128);patch([0 1 1 0],[0 0 1 1],c1);patch([0 1 1 1-e 1-e 0+e],[0 0 1 1-e 0+e 0+e],c2);patch([0 0 1 1-e 0+e 0+e],[0 1 1 1-e 1-e 0+e],c3);plot([0 1 1 0 0],[0 0 1 1 0]);
  Delays 1 : Subsystem
      mask Display: e = 0.06;c1 = [120 150 230]/255;c2 = ([120 150 230]+0)/383;c3 = ([120 150 230]+128)/383;patch([0 1 1 0],[0 0 1 1],c1);patch([0 1 1 1-e 1-e 0+e],[0 0 1 1-e 0+e 0+e],c2);patch([0 0 1 1-e 0+e 0+e],[0 1 1 1-e 1-e 0+e],c3);plot([0 1 1 0 0],[0 0 1 1 0]);disp('0');
  "IW{1,1}" : Subsystem
      mask Display: e = 0.06;c1 = [120 150 230]/255;c2 = ([120 150 230]+0)/383;c3 = ([120 150 230]+128)/383;patch([0 1 1 0],[0 0 1 1],c1);patch([0 1 1 1-e 1-e 0+e],[0 0 1 1-e 0+e 0+e],c2);patch([0 0 1 1-e 0+e 0+e],[0 1 1 1-e 1-e 0+e],c3);plot([0 1 1 0 0],[0 0 1 1 0]);disp('W');
  "b{1}" : Constant  Value=[-3.0166662633594057;1.0701809085177809;-1.6446607077141964;-0.55262743191566366;0.81692339434643979;-0.80237414732459966;0.76663591739284342;0.41098680957882483;-2.2933622794585817;-2.2588966761883844]
      mask Display: e = 0.06;c1 = [120 150 230]/255;c2 = ([120 150 230]+0)/383;c3 = ([120 150 230]+128)/383;patch([0 1 1 0],[0 0 1 1],c1);patch([0 1 1 1-e 1-e 0+e],[0 0 1 1-e 0+e 0+e],c2);patch([0 0 1 1-e 0+e 0+e],[0 1 1 1-e 1-e 0+e],c3);plot([0 1 1 0 0],[0 0 1 1 0]);disp('b');
  netsum : Sum  Inputs=2  SaturateOnIntegerOverflow=on  InputSameDT=on  OutDataTypeStr=Inherit: Same as first input
      mask Display: e = 0.06;c1 = [120 150 230]/255;c2 = ([120 150 230]+0)/383;c3 = ([120 150 230]+128)/383;patch([0 1 1 0],[0 0 1 1],c1);patch([0 1 1 1-e 1-e 0+e],[0 0 1 1-e 0+e 0+e],c2);patch([0 0 1 1-e 0+e 0+e],[0 1 1 1-e 1-e 0+e],c3);plot([0 1 1 0 0],[0 0 1 1 0]);disp('+');
  tansig : neural/Transfer Functions/tansig
  "a{1}" : Outport  InitialOutput=[0;0;0;0;0;0;0;0;0;0]
      mask Display: e = 0.06;c1 = [120 230 180]/255;c2 = ([120 230 180]+0)/(256+128);c3 = ([120 230 180]+128)/(256+128);patch([0 1 1 0],[0 0 1 1],c1);patch([0 1 1 1-e 1-e 0+e],[0 0 1 1-e 0+e 0+e],c2);patch([0 0 1 1-e 0+e 0+e],[0 1 1 1-e 1-e 0+e],c3);plot([0 1 1 0 0],[0 0 1 1 0]);
  wires:
  "p{1}"/1 -> Delays 1/1("p{1}")
  Delays 1/1("pd{1,1}") -> "IW{1,1}"/1("pd{1,1}")
  "IW{1,1}"/1("iz{1,1}") -> netsum/1
  "b{1}"/1 -> netsum/2
  netsum/1 -> tansig/1
  tansig/1 -> "a{1}"/1

== system AvonGasTurbineFAult/comp performance/Layer 2 ==
  "a{1} " : Inport  PortDimensions=10
      mask Display: e = 0.06;c1 = [120 230 180]/255;c2 = ([120 230 180]+0)/(256+128);c3 = ([120 230 180]+128)/(256+128);patch([0 1 1 0],[0 0 1 1],c1);patch([0 1 1 1-e 1-e 0+e],[0 0 1 1-e 0+e 0+e],c2);patch([0 0 1 1-e 0+e 0+e],[0 1 1 1-e 1-e 0+e],c3);plot([0 1 1 0 0],[0 0 1 1 0]);
  Delays 1 : Subsystem
      mask Display: e = 0.06;c1 = [120 150 230]/255;c2 = ([120 150 230]+0)/383;c3 = ([120 150 230]+128)/383;patch([0 1 1 0],[0 0 1 1],c1);patch([0 1 1 1-e 1-e 0+e],[0 0 1 1-e 0+e 0+e],c2);patch([0 0 1 1-e 0+e 0+e],[0 1 1 1-e 1-e 0+e],c3);plot([0 1 1 0 0],[0 0 1 1 0]);disp('0');
  "LW{2,1}" : Subsystem
      mask Display: e = 0.06;c1 = [120 150 230]/255;c2 = ([120 150 230]+0)/383;c3 = ([120 150 230]+128)/383;patch([0 1 1 0],[0 0 1 1],c1);patch([0 1 1 1-e 1-e 0+e],[0 0 1 1-e 0+e 0+e],c2);patch([0 0 1 1-e 0+e 0+e],[0 1 1 1-e 1-e 0+e],c3);plot([0 1 1 0 0],[0 0 1 1 0]);disp('W');
  "b{2}" : Constant  Value=[-1.7513533865709121;-0.36843921322469791;0.099194300057818097;0.34826117446019883;3.3782784836596536]
      mask Display: e = 0.06;c1 = [120 150 230]/255;c2 = ([120 150 230]+0)/383;c3 = ([120 150 230]+128)/383;patch([0 1 1 0],[0 0 1 1],c1);patch([0 1 1 1-e 1-e 0+e],[0 0 1 1-e 0+e 0+e],c2);patch([0 0 1 1-e 0+e 0+e],[0 1 1 1-e 1-e 0+e],c3);plot([0 1 1 0 0],[0 0 1 1 0]);disp('b');
  netsum : Sum  Inputs=2  SaturateOnIntegerOverflow=on  InputSameDT=on  OutDataTypeStr=Inherit: Same as first input
      mask Display: e = 0.06;c1 = [120 150 230]/255;c2 = ([120 150 230]+0)/383;c3 = ([120 150 230]+128)/383;patch([0 1 1 0],[0 0 1 1],c1);patch([0 1 1 1-e 1-e 0+e],[0 0 1 1-e 0+e 0+e],c2);patch([0 0 1 1-e 0+e 0+e],[0 1 1 1-e 1-e 0+e],c3);plot([0 1 1 0 0],[0 0 1 1 0]);disp('+');
  softmax : neural/Transfer Functions/softmax
  "a{2}" : Outport  InitialOutput=[0;0;0;0;0]
      mask Display: e = 0.06;c1 = [120 230 180]/255;c2 = ([120 230 180]+0)/(256+128);c3 = ([120 230 180]+128)/(256+128);patch([0 1 1 0],[0 0 1 1],c1);patch([0 1 1 1-e 1-e 0+e],[0 0 1 1-e 0+e 0+e],c2);patch([0 0 1 1-e 0+e 0+e],[0 1 1 1-e 1-e 0+e],c3);plot([0 1 1 0 0],[0 0 1 1 0]);
  wires:
  "a{1} "/1 -> Delays 1/1("p{2}")
  Delays 1/1("pd{2,1}") -> "LW{2,1}"/1("ad{2,1}")
  "LW{2,1}"/1("lz{2,1}") -> netsum/1
  "b{2}"/1 -> netsum/2
  netsum/1 -> softmax/1
  softmax/1 -> "a{2}"/1

== system AvonGasTurbineFAult/comp performance/Process Input 1 ==
  x : Inport  PortDimensions=6
      mask Display: e = 0.06;c1 = [120 230 180]/255;c2 = ([120 230 180]+0)/(256+128);c3 = ([120 230 180]+128)/(256+128);patch([0 1 1 0],[0 0 1 1],c1);patch([0 1 1 1-e 1-e 0+e],[0 0 1 1-e 0+e 0+e],c2);patch([0 0 1 1-e 0+e 0+e],[0 1 1 1-e 1-e 0+e],c3);plot([0 1 1 0 0],[0 0 1 1 0]);
  mapminmax : neural/Processing Functions/mapminmax  xmin=[-0.0099251436812934912;0;0;-2.7206457077544428;0;0]  xmax=[0.37230275618354725;62.920409543555763;26.300756094012741;13.627941217339298;30.663666242441877;1.0233056862835035]  ymin=-1  ymax=1
  p : Outport  PortDimensions=6
      mask Display: e = 0.06;c1 = [120 230 180]/255;c2 = ([120 230 180]+0)/(256+128);c3 = ([120 230 180]+128)/(256+128);patch([0 1 1 0],[0 0 1 1],c1);patch([0 1 1 1-e 1-e 0+e],[0 0 1 1-e 0+e 0+e],c2);patch([0 0 1 1-e 0+e 0+e],[0 1 1 1-e 1-e 0+e],c3);plot([0 1 1 0 0],[0 0 1 1 0]);
  wires:
  x/1 -> mapminmax/1
  mapminmax/1 -> p/1

== system AvonGasTurbineFAult/comp performance/Process Output 1 ==
  a : Inport  PortDimensions=5
      mask Display: e = 0.06;c1 = [120 230 180]/255;c2 = ([120 230 180]+0)/(256+128);c3 = ([120 230 180]+128)/(256+128);patch([0 1 1 0],[0 0 1 1],c1);patch([0 1 1 1-e 1-e 0+e],[0 0 1 1-e 0+e 0+e],c2);patch([0 0 1 1-e 0+e 0+e],[0 1 1 1-e 1-e 0+e],c3);plot([0 1 1 0 0],[0 0 1 1 0]);
  y : Outport  PortDimensions=5
      mask Display: e = 0.06;c1 = [120 230 180]/255;c2 = ([120 230 180]+0)/(256+128);c3 = ([120 230 180]+128)/(256+128);patch([0 1 1 0],[0 0 1 1],c1);patch([0 1 1 1-e 1-e 0+e],[0 0 1 1-e 0+e 0+e],c2);patch([0 0 1 1-e 0+e 0+e],[0 1 1 1-e 1-e 0+e],c3);plot([0 1 1 0 0],[0 0 1 1 0]);
  wires:
  a/1 -> y/1

== system AvonGasTurbineFAult/exhst temp turbine gg/Layer 1 ==
  "p{1}" : Inport  PortDimensions=4
      mask Display: e = 0.06;c1 = [120 230 180]/255;c2 = ([120 230 180]+0)/(256+128);c3 = ([120 230 180]+128)/(256+128);patch([0 1 1 0],[0 0 1 1],c1);patch([0 1 1 1-e 1-e 0+e],[0 0 1 1-e 0+e 0+e],c2);patch([0 0 1 1-e 0+e 0+e],[0 1 1 1-e 1-e 0+e],c3);plot([0 1 1 0 0],[0 0 1 1 0]);
  Delays 1 : Subsystem
      mask Display: e = 0.06;c1 = [120 150 230]/255;c2 = ([120 150 230]+0)/383;c3 = ([120 150 230]+128)/383;patch([0 1 1 0],[0 0 1 1],c1);patch([0 1 1 1-e 1-e 0+e],[0 0 1 1-e 0+e 0+e],c2);patch([0 0 1 1-e 0+e 0+e],[0 1 1 1-e 1-e 0+e],c3);plot([0 1 1 0 0],[0 0 1 1 0]);disp('0');
  "IW{1,1}" : Subsystem
      mask Display: e = 0.06;c1 = [120 150 230]/255;c2 = ([120 150 230]+0)/383;c3 = ([120 150 230]+128)/383;patch([0 1 1 0],[0 0 1 1],c1);patch([0 1 1 1-e 1-e 0+e],[0 0 1 1-e 0+e 0+e],c2);patch([0 0 1 1-e 0+e 0+e],[0 1 1 1-e 1-e 0+e],c3);plot([0 1 1 0 0],[0 0 1 1 0]);disp('W');
  "b{1}" : Constant  Value=[-0.36714433505719574;4.171957052168457;-1.7610679720239906;2.1955821867065644;-1.7361627653117517;0.89571232552353919;-3.7724969892838036;-1.4077208997705311;3.1301228479901151;-1.435337158107306]
      mask Display: e = 0.06;c1 = [120 150 230]/255;c2 = ([120 150 230]+0)/383;c3 = ([120 150 230]+128)/383;patch([0 1 1 0],[0 0 1 1],c1);patch([0 1 1 1-e 1-e 0+e],[0 0 1 1-e 0+e 0+e],c2);patch([0 0 1 1-e 0+e 0+e],[0 1 1 1-e 1-e 0+e],c3);plot([0 1 1 0 0],[0 0 1 1 0]);disp('b');
  netsum : Sum  Inputs=2  SaturateOnIntegerOverflow=on  InputSameDT=on  OutDataTypeStr=Inherit: Same as first input
      mask Display: e = 0.06;c1 = [120 150 230]/255;c2 = ([120 150 230]+0)/383;c3 = ([120 150 230]+128)/383;patch([0 1 1 0],[0 0 1 1],c1);patch([0 1 1 1-e 1-e 0+e],[0 0 1 1-e 0+e 0+e],c2);patch([0 0 1 1-e 0+e 0+e],[0 1 1 1-e 1-e 0+e],c3);plot([0 1 1 0 0],[0 0 1 1 0]);disp('+');
  tansig : neural/Transfer Functions/tansig
  "a{1}" : Outport  InitialOutput=[0;0;0;0;0;0;0;0;0;0]
      mask Display: e = 0.06;c1 = [120 230 180]/255;c2 = ([120 230 180]+0)/(256+128);c3 = ([120 230 180]+128)/(256+128);patch([0 1 1 0],[0 0 1 1],c1);patch([0 1 1 1-e 1-e 0+e],[0 0 1 1-e 0+e 0+e],c2);patch([0 0 1 1-e 0+e 0+e],[0 1 1 1-e 1-e 0+e],c3);plot([0 1 1 0 0],[0 0 1 1 0]);
  wires:
  "p{1}"/1 -> Delays 1/1("p{1}")
  Delays 1/1("pd{1,1}") -> "IW{1,1}"/1("pd{1,1}")
  "IW{1,1}"/1("iz{1,1}") -> netsum/1
  "b{1}"/1 -> netsum/2
  netsum/1 -> tansig/1
  tansig/1 -> "a{1}"/1

== system AvonGasTurbineFAult/exhst temp turbine gg/Layer 2 ==
  "a{1} " : Inport  PortDimensions=10
      mask Display: e = 0.06;c1 = [120 230 180]/255;c2 = ([120 230 180]+0)/(256+128);c3 = ([120 230 180]+128)/(256+128);patch([0 1 1 0],[0 0 1 1],c1);patch([0 1 1 1-e 1-e 0+e],[0 0 1 1-e 0+e 0+e],c2);patch([0 0 1 1-e 0+e 0+e],[0 1 1 1-e 1-e 0+e],c3);plot([0 1 1 0 0],[0 0 1 1 0]);
  Delays 1 : Subsystem
      mask Display: e = 0.06;c1 = [120 150 230]/255;c2 = ([120 150 230]+0)/383;c3 = ([120 150 230]+128)/383;patch([0 1 1 0],[0 0 1 1],c1);patch([0 1 1 1-e 1-e 0+e],[0 0 1 1-e 0+e 0+e],c2);patch([0 0 1 1-e 0+e 0+e],[0 1 1 1-e 1-e 0+e],c3);plot([0 1 1 0 0],[0 0 1 1 0]);disp('0');
  "LW{2,1}" : Subsystem
      mask Display: e = 0.06;c1 = [120 150 230]/255;c2 = ([120 150 230]+0)/383;c3 = ([120 150 230]+128)/383;patch([0 1 1 0],[0 0 1 1],c1);patch([0 1 1 1-e 1-e 0+e],[0 0 1 1-e 0+e 0+e],c2);patch([0 0 1 1-e 0+e 0+e],[0 1 1 1-e 1-e 0+e],c3);plot([0 1 1 0 0],[0 0 1 1 0]);disp('W');
  "b{2}" : Constant  Value=[-1.7639722134577072;-3.4721553945455366;-0.035323182127136671;-0.011147216834609504;4.9043883186030852]
      mask Display: e = 0.06;c1 = [120 150 230]/255;c2 = ([120 150 230]+0)/383;c3 = ([120 150 230]+128)/383;patch([0 1 1 0],[0 0 1 1],c1);patch([0 1 1 1-e 1-e 0+e],[0 0 1 1-e 0+e 0+e],c2);patch([0 0 1 1-e 0+e 0+e],[0 1 1 1-e 1-e 0+e],c3);plot([0 1 1 0 0],[0 0 1 1 0]);disp('b');
  netsum : Sum  Inputs=2  SaturateOnIntegerOverflow=on  InputSameDT=on  OutDataTypeStr=Inherit: Same as first input
      mask Display: e = 0.06;c1 = [120 150 230]/255;c2 = ([120 150 230]+0)/383;c3 = ([120 150 230]+128)/383;patch([0 1 1 0],[0 0 1 1],c1);patch([0 1 1 1-e 1-e 0+e],[0 0 1 1-e 0+e 0+e],c2);patch([0 0 1 1-e 0+e 0+e],[0 1 1 1-e 1-e 0+e],c3);plot([0 1 1 0 0],[0 0 1 1 0]);disp('+');
  softmax : neural/Transfer Functions/softmax
  "a{2}" : Outport  InitialOutput=[0;0;0;0;0]
      mask Display: e = 0.06;c1 = [120 230 180]/255;c2 = ([120 230 180]+0)/(256+128);c3 = ([120 230 180]+128)/(256+128);patch([0 1 1 0],[0 0 1 1],c1);patch([0 1 1 1-e 1-e 0+e],[0 0 1 1-e 0+e 0+e],c2);patch([0 0 1 1-e 0+e 0+e],[0 1 1 1-e 1-e 0+e],c3);plot([0 1 1 0 0],[0 0 1 1 0]);
  wires:
  "a{1} "/1 -> Delays 1/1("p{2}")
  Delays 1/1("pd{2,1}") -> "LW{2,1}"/1("ad{2,1}")
  "LW{2,1}"/1("lz{2,1}") -> netsum/1
  "b{2}"/1 -> netsum/2
  netsum/1 -> softmax/1
  softmax/1 -> "a{2}"/1

== system AvonGasTurbineFAult/exhst temp turbine gg/Process Input 1 ==
  x : Inport  PortDimensions=6
      mask Display: e = 0.06;c1 = [120 230 180]/255;c2 = ([120 230 180]+0)/(256+128);c3 = ([120 230 180]+128)/(256+128);patch([0 1 1 0],[0 0 1 1],c1);patch([0 1 1 1-e 1-e 0+e],[0 0 1 1-e 0+e 0+e],c2);patch([0 0 1 1-e 0+e 0+e],[0 1 1 1-e 1-e 0+e],c3);plot([0 1 1 0 0],[0 0 1 1 0]);
  mapminmax : neural/Processing Functions/mapminmax  xmin=[-0.10536173539736993;-11.752579477211384;-8.4719602751335401;-12.628699432343183]  xmax=[0;0;0;0]  ymin=-1  ymax=1
  removeconstantrows : neural/Processing Functions/removeconstantrows  inputSize=6  keep=[1 3 4 5]
  p : Outport  PortDimensions=4
      mask Display: e = 0.06;c1 = [120 230 180]/255;c2 = ([120 230 180]+0)/(256+128);c3 = ([120 230 180]+128)/(256+128);patch([0 1 1 0],[0 0 1 1],c1);patch([0 1 1 1-e 1-e 0+e],[0 0 1 1-e 0+e 0+e],c2);patch([0 0 1 1-e 0+e 0+e],[0 1 1 1-e 1-e 0+e],c3);plot([0 1 1 0 0],[0 0 1 1 0]);
  wires:
  x/1 -> removeconstantrows/1
  removeconstantrows/1 -> mapminmax/1
  mapminmax/1 -> p/1

== system AvonGasTurbineFAult/exhst temp turbine gg/Process Output 1 ==
  a : Inport  PortDimensions=5
      mask Display: e = 0.06;c1 = [120 230 180]/255;c2 = ([120 230 180]+0)/(256+128);c3 = ([120 230 180]+128)/(256+128);patch([0 1 1 0],[0 0 1 1],c1);patch([0 1 1 1-e 1-e 0+e],[0 0 1 1-e 0+e 0+e],c2);patch([0 0 1 1-e 0+e 0+e],[0 1 1 1-e 1-e 0+e],c3);plot([0 1 1 0 0],[0 0 1 1 0]);
  y : Outport  PortDimensions=5
      mask Display: e = 0.06;c1 = [120 230 180]/255;c2 = ([120 230 180]+0)/(256+128);c3 = ([120 230 180]+128)/(256+128);patch([0 1 1 0],[0 0 1 1],c1);patch([0 1 1 1-e 1-e 0+e],[0 0 1 1-e 0+e 0+e],c2);patch([0 0 1 1-e 0+e 0+e],[0 1 1 1-e 1-e 0+e],c3);plot([0 1 1 0 0],[0 0 1 1 0]);
  wires:
  a/1 -> y/1

== system AvonGasTurbineFAult/FG_valve/Layer 1/Delays 1 ==
  "p{1}" : Inport  PortDimensions=6
      mask Display: e = 0.06;c1 = [120 230 180]/255;c2 = ([120 230 180]+0)/(256+128);c3 = ([120 230 180]+128)/(256+128);patch([0 1 1 0],[0 0 1 1],c1);patch([0 1 1 1-e 1-e 0+e],[0 0 1 1-e 0+e 0+e],c2);patch([0 0 1 1-e 0+e 0+e],[0 1 1 1-e 1-e 0+e],c3);plot([0 1 1 0 0],[0 0 1 1 0]);
  mux : Mux  Inputs=1
      mask Display: e = 0.06;c1 = [120 150 230]/255;c2 = ([120 150 230]+0)/383;c3 = ([120 150 230]+128)/383;patch([0 1 1 0],[0 0 1 1],c1);patch([0 1 1 1-e 1-e 0+e],[0 0 1 1-e 0+e 0+e],c2);patch([0 0 1 1-e 0+e 0+e],[0 1 1 1-e 1-e 0+e],c3);plot([0 1 1 0 0],[0 0 1 1 0]);disp('Mux')
  "pd{1,1}" : Outport
      mask Display: e = 0.06;c1 = [120 230 180]/255;c2 = ([120 230 180]+0)/(256+128);c3 = ([120 230 180]+128)/(256+128);patch([0 1 1 0],[0 0 1 1],c1);patch([0 1 1 1-e 1-e 0+e],[0 0 1 1-e 0+e 0+e],c2);patch([0 0 1 1-e 0+e 0+e],[0 1 1 1-e 1-e 0+e],c3);plot([0 1 1 0 0],[0 0 1 1 0]);
  wires:
  "p{1}"/1 -> mux/1
  mux/1 -> "pd{1,1}"/1

== system AvonGasTurbineFAult/FG_valve/Layer 1/IW{1,1} ==
  "pd{1,1}" : Inport  PortDimensions=6
      mask Display: e = 0.06;c1 = [120 230 180]/255;c2 = ([120 230 180]+0)/(256+128);c3 = ([120 230 180]+128)/(256+128);patch([0 1 1 0],[0 0 1 1],c1);patch([0 1 1 1-e 1-e 0+e],[0 0 1 1-e 0+e 0+e],c2);patch([0 0 1 1-e 0+e 0+e],[0 1 1 1-e 1-e 0+e],c3);plot([0 1 1 0 0],[0 0 1 1 0]);
  "IW{1,1}(1,:)'" : Constant  Value=[-0.75693384564086952;-3.121764635077886;-0.54064692443434093;-1.1157048050788108;-2.8677818434941398;-0.86965168184717745]
      mask Display: e = 0.06;c1 = [120 150 230]/255;c2 = ([120 150 230]+0)/383;c3 = ([120 150 230]+128)/383;patch([0 1 1 0],[0 0 1 1],c1);patch([0 1 1 1-e 1-e 0+e],[0 0 1 1-e 0+e 0+e],c2);patch([0 0 1 1-e 0+e 0+e],[0 1 1 1-e 1-e 0+e],c3);plot([0 1 1 0 0],[0 0 1 1 0]);disp('Weights');
  "IW{1,1}(10,:)'" : Constant  Value=[0.51444075107217102;-0.97147204865894088;-0.76498279357008425;0.7839418266235002;1.2294438354508836;-1.0971389148087638]
      mask Display: e = 0.06;c1 = [120 150 230]/255;c2 = ([120 150 230]+0)/383;c3 = ([120 150 230]+128)/383;patch([0 1 1 0],[0 0 1 1],c1);patch([0 1 1 1-e 1-e 0+e],[0 0 1 1-e 0+e 0+e],c2);patch([0 0 1 1-e 0+e 0+e],[0 1 1 1-e 1-e 0+e],c3);plot([0 1 1 0 0],[0 0 1 1 0]);disp('Weights');
  "IW{1,1}(2,:)'" : Constant  Value=[0.92757492701520294;2.9775335180270854;0.43486606062648059;-0.23428499038093165;0.58125806565825255;1.163478233464958]
      mask Display: e = 0.06;c1 = [120 150 230]/255;c2 = ([120 150 230]+0)/383;c3 = ([120 150 230]+128)/383;patch([0 1 1 0],[0 0 1 1],c1);patch([0 1 1 1-e 1-e 0+e],[0 0 1 1-e 0+e 0+e],c2);patch([0 0 1 1-e 0+e 0+e],[0 1 1 1-e 1-e 0+e],c3);plot([0 1 1 0 0],[0 0 1 1 0]);disp('Weights');
  "IW{1,1}(3,:)'" : Constant  Value=[-0.75801890334332078;-1.2203930954277706;-0.10936662564978263;0.45841510316818312;1.4776460220824297;-0.23952134251679097]
      mask Display: e = 0.06;c1 = [120 150 230]/255;c2 = ([120 150 230]+0)/383;c3 = ([120 150 230]+128)/383;patch([0 1 1 0],[0 0 1 1],c1);patch([0 1 1 1-e 1-e 0+e],[0 0 1 1-e 0+e 0+e],c2);patch([0 0 1 1-e 0+e 0+e],[0 1 1 1-e 1-e 0+e],c3);plot([0 1 1 0 0],[0 0 1 1 0]);disp('Weights');
  "IW{1,1}(4,:)'" : Constant  Value=[0.01618632759502386;-2.1134441252683098;-0.41963389731544148;-0.96733214311771643;-1.5770022555127692;-1.9115115404547418]
      mask Display: e = 0.06;c1 = [120 150 230]/255;c2 = ([120 150 230]+0)/383;c3 = ([120 150 230]+128)/383;patch([0 1 1 0],[0 0 1 1],c1);patch([0 1 1 1-e 1-e 0+e],[0 0 1 1-e 0+e 0+e],c2);patch([0 0 1 1-e 0+e 0+e],[0 1 1 1-e 1-e 0+e],c3);plot([0 1 1 0 0],[0 0 1 1 0]);disp('Weights');
  "IW{1,1}(5,:)'" : Constant  Value=[-1.0811444149463625;-3.2742743596110588;-2.3657140266208265;-1.1232398206134711;-1.5074841366098044;-1.4459098150024652]
      mask Display: e = 0.06;c1 = [120 150 230]/255;c2 = ([120 150 230]+0)/383;c3 = ([120 150 230]+128)/383;patch([0 1 1 0],[0 0 1 1],c1);patch([0 1 1 1-e 1-e 0+e],[0 0 1 1-e 0+e 0+e],c2);patch([0 0 1 1-e 0+e 0+e],[0 1 1 1-e 1-e 0+e],c3);plot([0 1 1 0 0],[0 0 1 1 0]);disp('Weights');
  "IW{1,1}(6,:)'" : Constant  Value=[-2.2127987979170856;3.0609162328606474;0.83445025297389697;-3.1983078874690118;-0.44360233864052151;0.13215426986953979]
      mask Display: e = 0.06;c1 = [120 150 230]/255;c2 = ([120 150 230]+0)/383;c3 = ([120 150 230]+128)/383;patch([0 1 1 0],[0 0 1 1],c1);patch([0 1 1 1-e 1-e 0+e],[0 0 1 1-e 0+e 0+e],c2);patch([0 0 1 1-e 0+e 0+e],[0 1 1 1-e 1-e 0+e],c3);plot([0 1 1 0 0],[0 0 1 1 0]);disp('Weights');
  "IW{1,1}(7,:)'" : Constant  Value=[-3.0366565782190622;-2.3060460353020984;-1.7017453960485212;1.91252221169416;-0.63079836848576554;-0.26454483150503999]
      mask Display: e = 0.06;c1 = [120 150 230]/255;c2 = ([120 150 230]+0)/383;c3 = ([120 150 230]+128)/383;patch([0 1 1 0],[0 0 1 1],c1);patch([0 1 1 1-e 1-e 0+e],[0 0 1 1-e 0+e 0+e],c2);patch([0 0 1 1-e 0+e 0+e],[0 1 1 1-e 1-e 0+e],c3);plot([0 1 1 0 0],[0 0 1 1 0]);disp('Weights');
  "IW{1,1}(8,:)'" : Constant  Value=[2.0615527385883441;1.9083661684856645;1.4096091669416431;-2.0867124724463109;-0.48881246802567291;-0.2509436116433475]
      mask Display: e = 0.06;c1 = [120 150 230]/255;c2 = ([120 150 230]+0)/383;c3 = ([120 150 230]+128)/383;patch([0 1 1 0],[0 0 1 1],c1);patch([0 1 1 1-e 1-e 0+e],[0 0 1 1-e 0+e 0+e],c2);patch([0 0 1 1-e 0+e 0+e],[0 1 1 1-e 1-e 0+e],c3);plot([0 1 1 0 0],[0 0 1 1 0]);disp('Weights');
  "IW{1,1}(9,:)'" : Constant  Value=[3.7646727642987989;3.6036237647988179;2.321866995571185;-0.75607253792316254;0.903729227894006;0.44957483484425753]
      mask Display: e = 0.06;c1 = [120 150 230]/255;c2 = ([120 150 230]+0)/383;c3 = ([120 150 230]+128)/383;patch([0 1 1 0],[0 0 1 1],c1);patch([0 1 1 1-e 1-e 0+e],[0 0 1 1-e 0+e 0+e],c2);patch([0 0 1 1-e 0+e 0+e],[0 1 1 1-e 1-e 0+e],c3);plot([0 1 1 0 0],[0 0 1 1 0]);disp('Weights');
  Mux : Mux  Inputs=10
      mask Display: e = 0.06;c1 = [120 150 230]/255;c2 = ([120 150 230]+0)/383;c3 = ([120 150 230]+128)/383;patch([0 1 1 0],[0 0 1 1],c1);patch([0 1 1 1-e 1-e 0+e],[0 0 1 1-e 0+e 0+e],c2);patch([0 0 1 1-e 0+e 0+e],[0 1 1 1-e 1-e 0+e],c3);plot([0 1 1 0 0],[0 0 1 1 0]);disp('Mux');
  dotprod{1..10} (10 alike) : neural/Weight Functions/dotprod
  "iz{1,1}" : Outport
      mask Display: e = 0.06;c1 = [120 230 180]/255;c2 = ([120 230 180]+0)/(256+128);c3 = ([120 230 180]+128)/(256+128);patch([0 1 1 0],[0 0 1 1],c1);patch([0 1 1 1-e 1-e 0+e],[0 0 1 1-e 0+e 0+e],c2);patch([0 0 1 1-e 0+e 0+e],[0 1 1 1-e 1-e 0+e],c3);plot([0 1 1 0 0],[0 0 1 1 0]);
  wires:
  "IW{1,1}(1,:)'"/1 -> dotprod1/1
  "pd{1,1}"/1 -> dotprod1/2, dotprod2/2, dotprod3/2, dotprod4/2, dotprod5/2, dotprod6/2, dotprod7/2, dotprod8/2, dotprod9/2, dotprod10/2
  dotprod1/1 -> Mux/1
  "IW{1,1}(2,:)'"/1 -> dotprod2/1
  dotprod2/1 -> Mux/2
  "IW{1,1}(3,:)'"/1 -> dotprod3/1
  dotprod3/1 -> Mux/3
  "IW{1,1}(4,:)'"/1 -> dotprod4/1
  dotprod4/1 -> Mux/4
  "IW{1,1}(5,:)'"/1 -> dotprod5/1
  dotprod5/1 -> Mux/5
  "IW{1,1}(6,:)'"/1 -> dotprod6/1
  dotprod6/1 -> Mux/6
  "IW{1,1}(7,:)'"/1 -> dotprod7/1
  dotprod7/1 -> Mux/7
  "IW{1,1}(8,:)'"/1 -> dotprod8/1
  dotprod8/1 -> Mux/8
  "IW{1,1}(9,:)'"/1 -> dotprod9/1
  dotprod9/1 -> Mux/9
  "IW{1,1}(10,:)'"/1 -> dotprod10/1
  dotprod10/1 -> Mux/10
  Mux/1 -> "iz{1,1}"/1

== system AvonGasTurbineFAult/FG_valve/Layer 2/Delays 1 ==
  "p{2}" : Inport  PortDimensions=10
      mask Display: e = 0.06;c1 = [120 230 180]/255;c2 = ([120 230 180]+0)/(256+128);c3 = ([120 230 180]+128)/(256+128);patch([0 1 1 0],[0 0 1 1],c1);patch([0 1 1 1-e 1-e 0+e],[0 0 1 1-e 0+e 0+e],c2);patch([0 0 1 1-e 0+e 0+e],[0 1 1 1-e 1-e 0+e],c3);plot([0 1 1 0 0],[0 0 1 1 0]);
  mux : Mux  Inputs=1
      mask Display: e = 0.06;c1 = [120 150 230]/255;c2 = ([120 150 230]+0)/383;c3 = ([120 150 230]+128)/383;patch([0 1 1 0],[0 0 1 1],c1);patch([0 1 1 1-e 1-e 0+e],[0 0 1 1-e 0+e 0+e],c2);patch([0 0 1 1-e 0+e 0+e],[0 1 1 1-e 1-e 0+e],c3);plot([0 1 1 0 0],[0 0 1 1 0]);disp('Mux')
  "pd{2,1}" : Outport
      mask Display: e = 0.06;c1 = [120 230 180]/255;c2 = ([120 230 180]+0)/(256+128);c3 = ([120 230 180]+128)/(256+128);patch([0 1 1 0],[0 0 1 1],c1);patch([0 1 1 1-e 1-e 0+e],[0 0 1 1-e 0+e 0+e],c2);patch([0 0 1 1-e 0+e 0+e],[0 1 1 1-e 1-e 0+e],c3);plot([0 1 1 0 0],[0 0 1 1 0]);
  wires:
  "p{2}"/1 -> mux/1
  mux/1 -> "pd{2,1}"/1
